simulink model "bicycle_3dof"  (R2026b)
settings: Solver=VariableStepAuto
undefined symbols (not defined in the file): Params
settings Model: Creator=andrei  LastModifiedBy=andrei

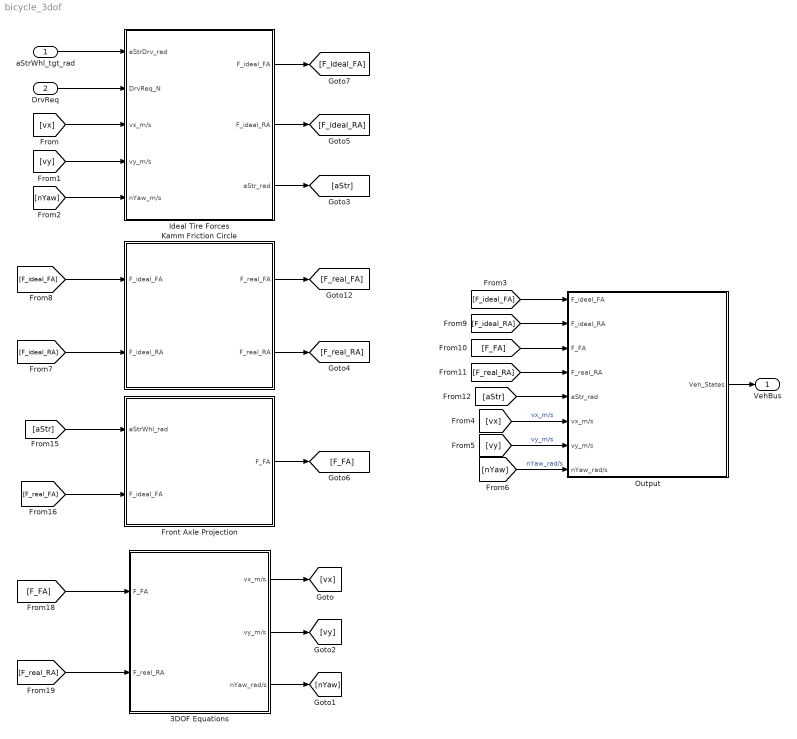
== system bicycle_3dof ==
  aStrWhl_tgt_rad : Inport
  DrvReq : Inport  Port=2
  3DOF Equations : Subsystem
  Front Axle Projection : Subsystem
  Ideal Tire Forces : Subsystem
  Kamm Friction Circle : Subsystem
  Output : Subsystem
  VehBus : Outport
  wires:
  [aStr] -> Front Axle Projection/1(aStrWhl_rad)
  [vy] -> Ideal Tire Forces/4(vy_m/s)
  3DOF Equations/2(vy_m/s) -> [vy]
  3DOF Equations/3(nYaw_rad/s) -> [nYaw]
  3DOF Equations/1(vx_m/s) -> [vx]
  [vx] -> Ideal Tire Forces/3(vx_m/s)
  [nYaw] -> Ideal Tire Forces/5(nYaw_m/s)
  [F_ideal_FA] -> Kamm Friction Circle/1(F_ideal_FA)
  [F_real_FA] -> Front Axle Projection/2(F_ideal_FA)
  [F_FA] -> 3DOF Equations/1(F_FA)
  [F_ideal_RA] -> Kamm Friction Circle/2(F_ideal_RA)
  DrvReq/1 -> Ideal Tire Forces/2(DrvReq_N)
  [F_real_RA] -> 3DOF Equations/2(F_real_RA)
  aStrWhl_tgt_rad/1 -> Ideal Tire Forces/1(aStrDrv_rad)
  Kamm Friction Circle/1(F_real_FA) -> [F_real_FA]
  Ideal Tire Forces/3(aStr_rad) -> [aStr]
  Kamm Friction Circle/2(F_real_RA) -> [F_real_RA]
  Front Axle Projection/1(F_FA) -> [F_FA]
  Ideal Tire Forces/1(F_ideal_FA) -> [F_ideal_FA]
  Ideal Tire Forces/2(F_ideal_RA) -> [F_ideal_RA]
  [F_ideal_FA] -> Output/1(F_ideal_FA)
  [F_ideal_RA] -> Output/2(F_ideal_RA)
  [F_FA] -> Output/3(F_FA)
  [F_real_RA] -> Output/4(F_real_RA)
  [aStr] -> Output/5(aStr_rad)
  [vx] -> Output/6(vx_m/s)  "vx_m/s"
  [vy] -> Output/7(vy_m/s)  "vy_m/s"
  [nYaw] -> Output/8(nYaw_rad/s)  "nYaw_rad/s"
  Output/1(Veh_States) -> VehBus/1

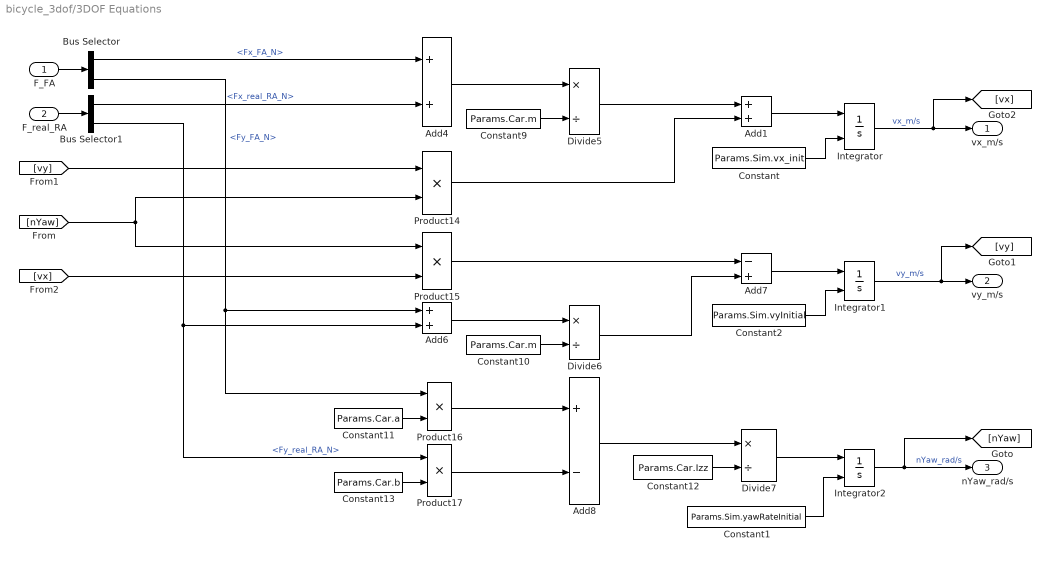
== system bicycle_3dof/3DOF Equations ==
  F_FA : Inport
  F_real_RA : Inport  Port=2
  Add1 : Sum
  Add4 : Sum
  Add6 : Sum
  Add7 : Sum  Inputs=-+
  Add8 : Sum  Inputs=+-
  Bus Selector : BusSelector  OutputSignals=Fx_FA_N,Fy_FA_N
  Bus Selector1 : BusSelector  OutputSignals=Fx_real_RA_N,Fy_real_RA_N
  Constant : Constant  Value=Params.Sim.vx_init
  Constant1 : Constant  Value=Params.Sim.yawRateInitial
  Constant10 : Constant  Value=Params.Car.m
  Constant11 : Constant  Value=Params.Car.a
  Constant12 : Constant  Value=Params.Car.Izz
  Constant13 : Constant  Value=Params.Car.b
  Constant2 : Constant  Value=Params.Sim.vyInitial
  Constant9 : Constant  Value=Params.Car.m
  Divide5 : Product  Inputs=*/
  Divide6 : Product  Inputs=*/
  Divide7 : Product  Inputs=*/
  Integrator : Integrator  InitialConditionSource=external  InitialCondition=Params.Sim.vx_init  LimitOutput=on  UpperSaturationLimit=Params.Sim.vxMax  LowerSaturationLimit=Params.Sim.vxMin
  Integrator1 : Integrator  InitialConditionSource=external  InitialCondition=Params.Sim.vyInitial  LimitOutput=on  UpperSaturationLimit=Params.Sim.vyMaxAbs  LowerSaturationLimit=-Params.Sim.vyMaxAbs
  Integrator2 : Integrator  InitialConditionSource=external  InitialCondition=Params.Sim.yawRateInitial
  Product{14..17} (4 alike) : Product
  vx_m/s : Outport
  vy_m/s : Outport  Port=2
  nYaw_rad/s : Outport  Port=3
  wires:
  [nYaw] -> Product15/1, Product14/2
  Constant1/1 -> Integrator2/2
  Constant2/1 -> Integrator1/2
  Constant/1 -> Integrator/2
  Bus Selector/2 -> Add6/1, Product16/1  "<Fy_FA_N>"
  Bus Selector1/1 -> Add4/2  "<Fx_real_RA_N>"
  Bus Selector/1 -> Add4/1  "<Fx_FA_N>"
  Integrator/1 -> vx_m/s/1, [vx]  "vx_m/s"
  Integrator1/1 -> vy_m/s/1, [vy]  "vy_m/s"
  F_real_RA/1 -> Bus Selector1/1
  F_FA/1 -> Bus Selector/1
  Constant13/1 -> Product17/2
  Divide7/1 -> Integrator2/1
  Add8/1 -> Divide7/1
  Product16/1 -> Add8/1
  Product17/1 -> Add8/2
  [vy] -> Product14/1
  Product15/1 -> Add7/1
  Bus Selector1/2 -> Add6/2, Product17/1  "<Fy_real_RA_N>"
  Add7/1 -> Integrator1/1
  Constant10/1 -> Divide6/2
  Divide6/1 -> Add7/2
  Constant11/1 -> Product16/2
  Add6/1 -> Divide6/1
  Add1/1 -> Integrator/1
  Integrator2/1 -> [nYaw], nYaw_rad/s/1  "nYaw_rad/s"
  [vx] -> Product15/2
  Product14/1 -> Add1/2
  Constant12/1 -> Divide7/2
  Add4/1 -> Divide5/1
  Divide5/1 -> Add1/1
  Constant9/1 -> Divide5/2

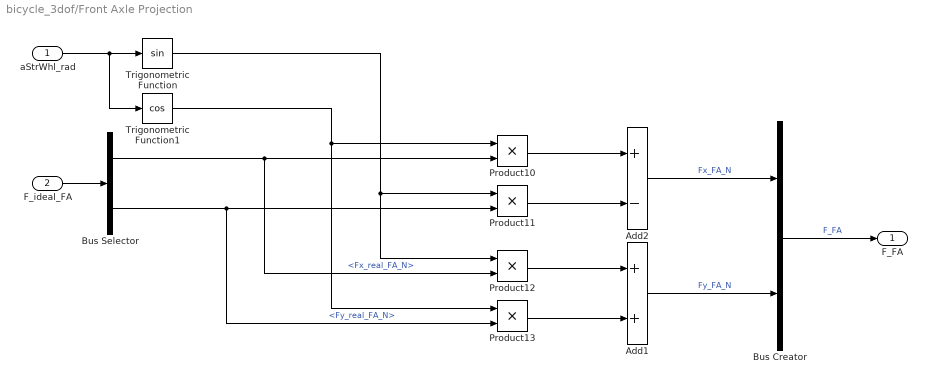
== system bicycle_3dof/Front Axle Projection ==
  aStrWhl_rad : Inport
  F_ideal_FA : Inport  Port=2
  Add1 : Sum
  Add2 : Sum  Inputs=+-
  Bus Creator : BusCreator  Inputs=2
  Bus Selector : BusSelector  OutputSignals=Fx_real_FA_N,Fy_real_FA_N
  Product{10..13} (4 alike) : Product
  Trigonometric Function : Trigonometry
  Trigonometric Function1 : Trigonometry  Operator=cos
  F_FA : Outport
  wires:
  Bus Creator/1 -> F_FA/1  "F_FA"
  F_ideal_FA/1 -> Bus Selector/1
  Add1/1 -> Bus Creator/2  "Fy_FA_N"
  Add2/1 -> Bus Creator/1  "Fx_FA_N"
  Product13/1 -> Add1/2
  Product11/1 -> Add2/2
  Product12/1 -> Add1/1
  Trigonometric Function/1 -> Product11/1, Product12/1
  Trigonometric Function1/1 -> Product10/1, Product13/1
  Product10/1 -> Add2/1
  Bus Selector/1 -> Product10/2, Product12/2  "<Fx_real_FA_N>"
  Bus Selector/2 -> Product13/2, Product11/2  "<Fy_real_FA_N>"
  aStrWhl_rad/1 -> Trigonometric Function/1, Trigonometric Function1/1

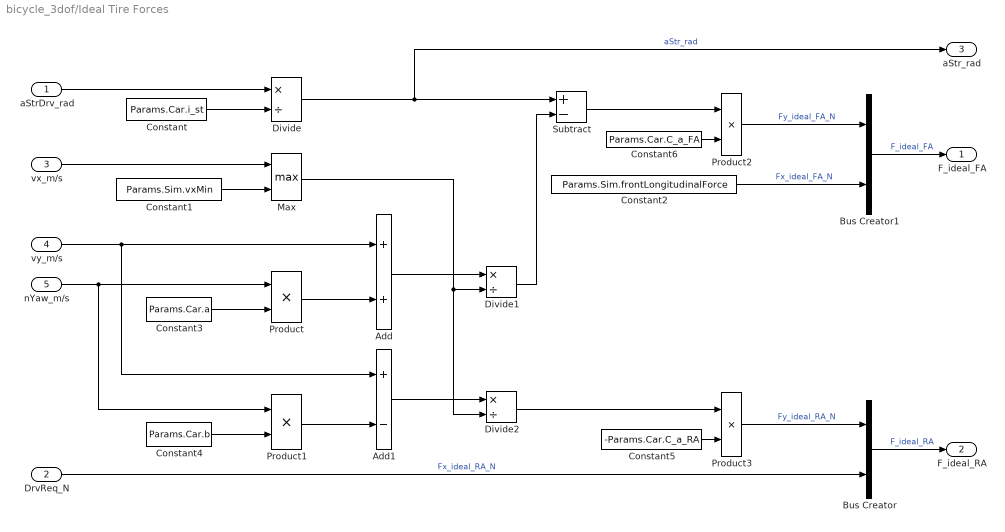
== system bicycle_3dof/Ideal Tire Forces ==
  aStrDrv_rad : Inport
  DrvReq_N : Inport  Port=2
  vx_m/s : Inport  Port=3
  vy_m/s : Inport  Port=4
  nYaw_m/s : Inport  Port=5
  Add : Sum
  Add1 : Sum  Inputs=+-
  Bus Creator : BusCreator  Inputs=2
  Bus Creator1 : BusCreator  Inputs=2
  Constant : Constant  Value=Params.Car.i_st
  Constant1 : Constant  Value=Params.Sim.vxMin
  Constant2 : Constant  Value=Params.Sim.frontLongitudinalForce
  Constant3 : Constant  Value=Params.Car.a
  Constant4 : Constant  Value=Params.Car.b
  Constant5 : Constant  Value=-Params.Car.C_a_RA
  Constant6 : Constant  Value=Params.Car.C_a_FA
  Divide : Product  Inputs=*/
  Divide1 : Product  Inputs=*/
  Divide2 : Product  Inputs=*/
  Max : MinMax  Function=max  Inputs=2
  Product{,1..3} (4 alike) : Product
  Subtract : Sum  Inputs=+-
  F_ideal_FA : Outport
  F_ideal_RA : Outport  Port=2
  aStr_rad : Outport  Port=3
  wires:
  Bus Creator1/1 -> F_ideal_FA/1  "F_ideal_FA"
  DrvReq_N/1 -> Bus Creator/2  "Fx_ideal_RA_N"
  Bus Creator/1 -> F_ideal_RA/1  "F_ideal_RA"
  Divide/1 -> Subtract/1, aStr_rad/1  "aStr_rad"
  Constant2/1 -> Bus Creator1/2  "Fx_ideal_FA_N"
  Subtract/1 -> Product2/1
  Max/1 -> Divide1/2, Divide2/2
  Constant1/1 -> Max/2
  vx_m/s/1 -> Max/1
  Product3/1 -> Bus Creator/1  "Fy_ideal_RA_N"
  Product2/1 -> Bus Creator1/1  "Fy_ideal_FA_N"
  Constant4/1 -> Product1/2
  Product1/1 -> Add1/2
  aStrDrv_rad/1 -> Divide/1
  Add1/1 -> Divide2/1
  Constant3/1 -> Product/2
  Product/1 -> Add/2
  Constant5/1 -> Product3/2
  Divide2/1 -> Product3/1
  nYaw_m/s/1 -> Product/1, Product1/1
  Divide1/1 -> Subtract/2
  vy_m/s/1 -> Add/1, Add1/1
  Add/1 -> Divide1/1
  Constant6/1 -> Product2/2
  Constant/1 -> Divide/2

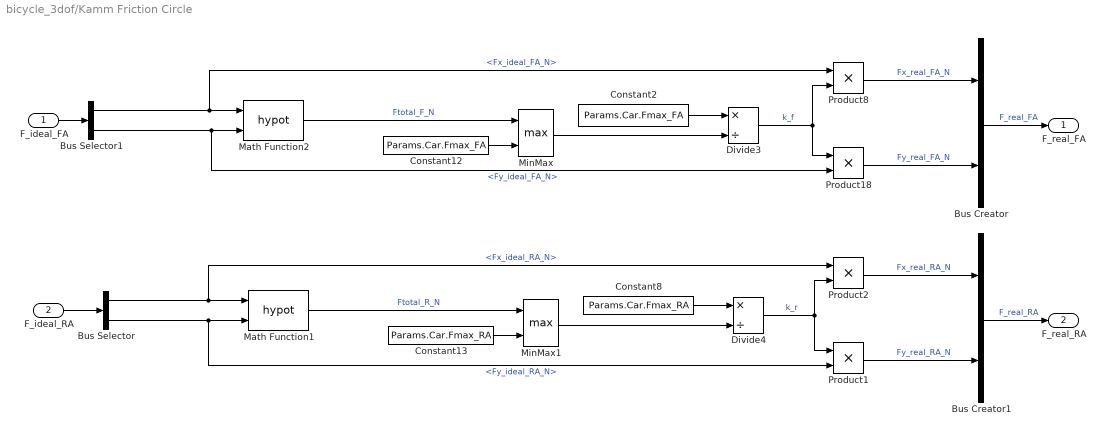
== system bicycle_3dof/Kamm Friction Circle ==
  F_ideal_FA : Inport
  F_ideal_RA : Inport  Port=2
  Bus Creator : BusCreator  Inputs=2
  Bus Creator1 : BusCreator  Inputs=2
  Bus Selector : BusSelector  OutputSignals=Fx_ideal_RA_N,Fy_ideal_RA_N
  Bus Selector1 : BusSelector  OutputSignals=Fx_ideal_FA_N,Fy_ideal_FA_N
  Constant12 : Constant  Value=Params.Car.Fmax_FA
  Constant13 : Constant  Value=Params.Car.Fmax_RA
  Constant2 : Constant  Value=Params.Car.Fmax_FA
  Constant8 : Constant  Value=Params.Car.Fmax_RA
  Divide3 : Product  Inputs=*/
  Divide4 : Product  Inputs=*/
  Math Function1 : Math  Operator=hypot
  Math Function2 : Math  Operator=hypot
  MinMax : MinMax  Function=max  Inputs=2
  MinMax1 : MinMax  Function=max  Inputs=2
  Product{1..2,8,18} (4 alike) : Product
  F_real_FA : Outport
  F_real_RA : Outport  Port=2
  wires:
  Bus Creator1/1 -> F_real_RA/1  "F_real_RA"
  Product1/1 -> Bus Creator1/2  "Fy_real_RA_N"
  Product2/1 -> Bus Creator1/1  "Fx_real_RA_N"
  Bus Creator/1 -> F_real_FA/1  "F_real_FA"
  Bus Selector/2 -> Math Function1/2, Product1/2  "<Fy_ideal_RA_N>"
  Bus Selector/1 -> Product2/1, Math Function1/1  "<Fx_ideal_RA_N>"
  Bus Selector1/2 -> Math Function2/2, Product18/2  "<Fy_ideal_FA_N>"
  Bus Selector1/1 -> Math Function2/1, Product8/1  "<Fx_ideal_FA_N>"
  F_ideal_FA/1 -> Bus Selector1/1
  F_ideal_RA/1 -> Bus Selector/1
  Math Function2/1 -> MinMax/1  "Ftotal_F_N"
  Constant13/1 -> MinMax1/2
  MinMax1/1 -> Divide4/2
  Math Function1/1 -> MinMax1/1  "Ftotal_R_N"
  Divide4/1 -> Product2/2, Product1/1  "k_r"
  MinMax/1 -> Divide3/2
  Constant2/1 -> Divide3/1
  Product18/1 -> Bus Creator/2  "Fy_real_FA_N"
  Divide3/1 -> Product8/2, Product18/1  "k_f"
  Product8/1 -> Bus Creator/1  "Fx_real_FA_N"
  Constant8/1 -> Divide4/1
  Constant12/1 -> MinMax/2

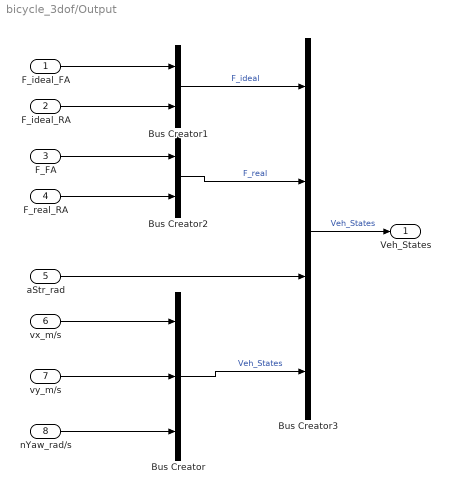
== system bicycle_3dof/Output ==
  F_ideal_FA : Inport
  F_ideal_RA : Inport  Port=2
  F_FA : Inport  Port=3
  F_real_RA : Inport  Port=4
  aStr_rad : Inport  Port=5
  vx_m/s : Inport  Port=6
  vy_m/s : Inport  Port=7
  nYaw_rad/s : Inport  Port=8
  Bus Creator : BusCreator  Inputs=3
  Bus Creator1 : BusCreator  Inputs=2
  Bus Creator2 : BusCreator  Inputs=2
  Bus Creator3 : BusCreator  Inputs=4
  Veh_States : Outport
  wires:
  aStr_rad/1 -> Bus Creator3/3
  Bus Creator/1 -> Bus Creator3/4  "Veh_States"
  F_FA/1 -> Bus Creator2/1
  vy_m/s/1 -> Bus Creator/2
  F_ideal_FA/1 -> Bus Creator1/1
  Bus Creator2/1 -> Bus Creator3/2  "F_real"
  vx_m/s/1 -> Bus Creator/1
  F_ideal_RA/1 -> Bus Creator1/2
  Bus Creator3/1 -> Veh_States/1  "Veh_States"
  Bus Creator1/1 -> Bus Creator3/1  "F_ideal"
  F_real_RA/1 -> Bus Creator2/2
  nYaw_rad/s/1 -> Bus Creator/3
